simulink model "viikate_rocket"  (R2026b)
settings: Solver=ode4  StopTime=inf  FixedStep=0.001
undefined symbols (not defined in the file or in its folder): Aero, e0_0, e1_0, e2_0, e3_0, gravity, I, N, Newton, Raphson, rho, rp_burn_time_s, rp_canard_area_m2, rp_canard_cl_alpha, rp_cd0, rp_clp, rp_cmq, rp_cn_alpha, rp_cnr, rp_fin_positions_m, rp_frontal_area_m2, rp_gust_seed, rp_gust_variance, rp_ignition_time_s, rp_inertia_empty_kgm2, rp_inertia_full_kgm2, rp_length_m, rp_mass_fuel_kg, rp_mass_full_kg, rp_r_cp_m, rp_roll_ref_length_m, rp_servo_rate_limit_radps, rp_servo_tau_s, rp_thrust_n, rp_thrust_scale, rp_thrust_t_s, rp_wind_model_mps, sharedaeroassertmsg, si, Vsafe, ZYX
libraries: matrix_library x1
(part 3 of 3)

== system viikate_rocket/Simple Variable Mass 6DOF/Calculate DCM & Euler Angles/Quaternions to Rotation Angles/DCM2Ang/Validate DCM/If Warning//Error/isNotProper/determinant does not equal 1 ==
  u : Inport
  Compare : RelationalOperator  Operator=>  OutDataTypeStr=boolean
  Constant : Constant  DisableCoverage=on  Value=const  OutDataTypeStr=Inherit: Inherit via back propagation
  y : Outport
  wires:
  u/1 -> Compare/1
  Constant/1 -> Compare/2
  Compare/1 -> y/1

== matlab function viikate_rocket/aerodynamics/Canard fin forces/MATLAB Function1 ==
  data: L input; F output; N input
function F = scaleForces(L,N)

F = L .* N;

end

== matlab function viikate_rocket/aerodynamics/Canard fin forces/MATLAB Function ==
  data: r input; M output; F input
function M = computeTorque(r,F)

M = [0 0 0];

for i = 1:4
    M = M + cross(r(i,:), F(i,:));
end

end

== matlab function viikate_rocket/aerodynamics/Canard fin forces/MATLAB Function2 ==
  data: a input; ci output
function ci = chordDirections(a)
    ci = [cos(a(1)) sin(a(1)) 0; cos(a(2)) 0 sin(a(2)); cos(a(3)) -sin(a(3)) 0; cos(a(4)) 0 -sin(a(4))];
end

== matlab function viikate_rocket/aerodynamics/Canard fin forces/MATLAB Function3 ==
  data: si input; ni output; ci input
function ni = fcn(si, ci)
    ni = cross(si, ci);
end

== matlab function viikate_rocket/aerodynamics/Canard fin forces/MATLAB Function4 ==
  data: FN input; finForces output
function finForces = fcn(FN)
    finForces = sum(FN,1)';
end
